simulink model "FullFMS_SIM_V0_1_7_R2026a"  (R2026a)
settings: Solver=FixedStepAuto  StopTime=inf  FixedStep=0.01  MaxStep=0.01  RelTol=1e-2
PreLoadFcn:
  | load("BUS_CONFIG_SIM.mat"); run("Param_SIM_V0_1_7.m")
libraries: opcualib x8
(part 1 of 2)
settings Model: SimulationMode=accelerator  PacingRate=0.100000  Creator=guilh  LastModifiedBy=gasie
settings SolverCC: ZeroCrossControl=DisableAll

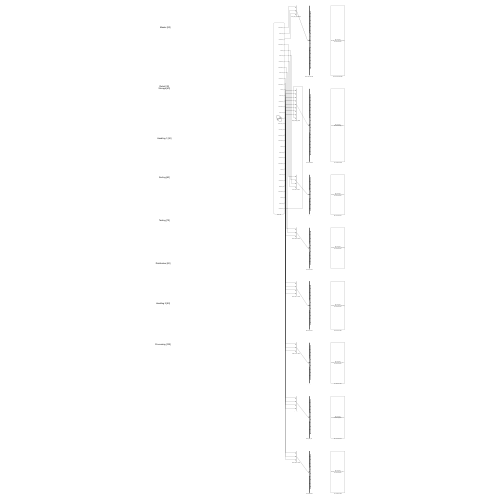
[thumbnail: Simulink's stored preview of the top-level diagram]
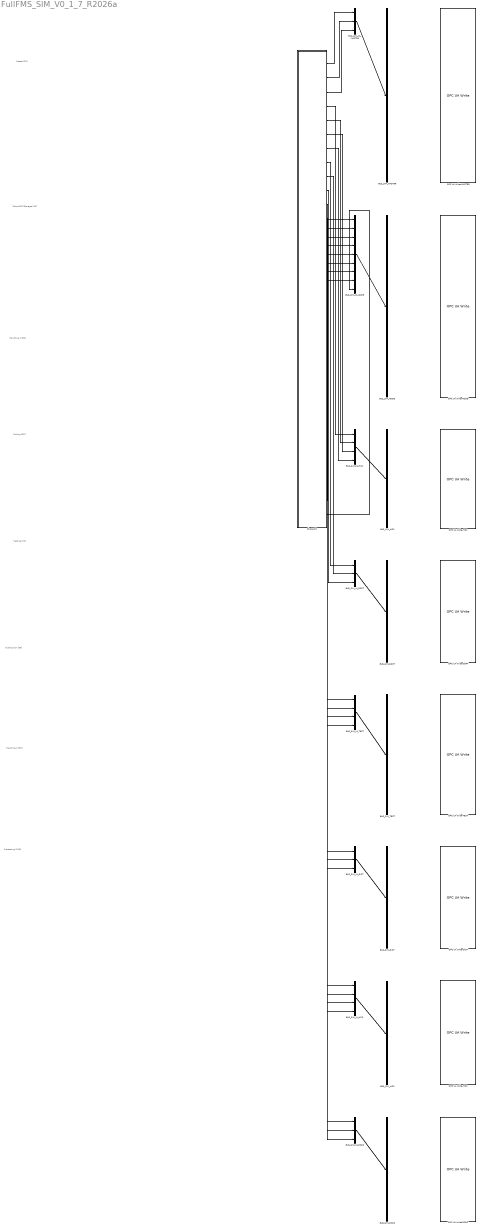
== system FullFMS_SIM_V0_1_7_R2026a ==
  note: Master [20]
  note: Robot [30]
      | Storage [40]
  note: Handling 1 [50]
  note: Sorting [60]
  note: Testing [70]
  note: Distribution [80]
  note: Handling 2 [90]
  note: Processing [100]
  BUS_SIM_DIST : BusSelector  OutputSignals=SimActuators_80.SA_80_Pist_Adv,SimActuators_80.SA_80_Suction_On,SimActuators_80.SA_80_Suction_Off,SimActuators_80.SA_80_Arm_2_Del,SimActuators_80.SA_80_Arm_2_Mag,SimActuators_80.SA_81_Led_Start,SimActuators_80.SA_81_Led_Reset,SimActuators_80.SA_81_Led_Extra1,SimActuators_80.SA_81_Led_Extra2,SimActuators_80.SA_81_Panel_O4,SimActuators_80.SA_81_Panel_O5,SimActuators_80.SA_81_Panel_O6,SimActuators_80.SA_81_Panel_O7,SimControl_80.SC_82_Profibus,SimControl_80.SC_83_RQ_Parts,SimControl_80.SC_85_Initialization,SimControl_80.SC_85_Start,SimControl_80.SC_85_Part_Del,SimControl_80.SC_85_Single,SimControl_80.SC_85_Part_Mag,SimControl_80.SC_85_Continuous,SimControl_80.SC_85_Counted,SimControl_80.SC_86_Mag_Parts,SimControl_80.SC_87_RQ_MParts,SimSensors_80.SS_80_Mag_Full,SimSensors_80.SS_80_Pist_Bck,SimSensors_80.SS_80_Pist_Fwd,SimSensors_80.SS_80_Part_Stuck,SimSensors_80.SS_80_Arm_Mag,SimSensors_80.SS_80_Arm_Del,SimSensors_80.SS_80_Mag_Empty,SimSensors_80.SS_81_Start,SimSensors_80.SS_81_Stop,SimSensors_80.SS_81_Key_Pos,SimSensors_80.SS_81_Reset,SimSensors_80.SS_81_Panel_I4,SimSensors_80.SS_81_Panel_I5,SimSensors_80.SS_81_Panel_I6,SimSensors_80.SS_81_Panel_I7
  BUS_SIM_HD1 : BusSelector  OutputSignals=SimActuators_50.SA_50_Claw_2_Del,SimActuators_50.SA_50_Claw_2_Cart,SimActuators_50.SA_50_Claw_Down,SimActuators_50.SA_50_Close_Claw,SimActuators_50.SA_51_Led_Start,SimActuators_50.SA_51_Led_Reset,SimActuators_50.SA_51_Led_Extra1,SimActuators_50.SA_51_Led_Extra2,SimActuators_50.SA_51_Panel_O4,SimActuators_50.SA_51_Panel_O5,SimActuators_50.SA_51_Panel_O6,SimActuators_50.SA_51_Panel_O7,SimASi_50.SR_53_SortCartID,SimASi_50.SR_54_Request,SimASi_50.SR_54_No_Cart,SimASi_50.SR_54_Cart_Full,SimASi_50.SR_54_CRoute_Out,SimASi_50.SR_54_CRoute_In,SimControl_50.SC_52_Profibus,SimControl_50.SC_55_Initialization,SimControl_50.SC_55_Start,SimControl_50.SC_55_PD_Sort,SimControl_50.SC_55_Cart2Del,SimSensors_50.SS_50_Part_Reserve,SimSensors_50.SS_50_Claw_Cart,SimSensors_50.SS_50_Claw_Del,SimSensors_50.SS_50_Claw_Reserve,SimSensors_50.SS_50_Claw_Low,SimSensors_50.SS_50_Claw_High,SimSensors_50.SS_50_Part_in_Claw,SimSensors_50.SS_51_Start,SimSensors_50.SS_51_Stop,SimSensors_50.SS_51_Key_Pos,SimSensors_50.SS_51_Reset,SimSensors_50.SS_51_Panel_I4,SimSensors_50.SS_51_Panel_I5,SimSensors_50.SS_51_Panel_I6,SimSensors_50.SS_51_Panel_I7
  BUS_SIM_HD2 : BusSelector  OutputSignals=SimActuators_90.SA_90_Claw_2_Cart,SimActuators_90.SA_90_Claw_2_Del,SimActuators_90.SA_90_Claw_Down,SimActuators_90.SA_90_Close_Claw,SimActuators_90.SA_91_Led_Start,SimActuators_90.SA_91_Led_Reset,SimActuators_90.SA_91_Led_Extra1,SimActuators_90.SA_91_Led_Extra2,SimActuators_90.SA_91_Panel_O4,SimActuators_90.SA_91_Panel_O5,SimActuators_90.SA_91_Panel_O6,SimActuators_90.SA_91_Panel_O7,SimASi_90.SR_93_ProcCartID,SimASi_90.SR_94_Request,SimASi_90.SR_94_No_Cart,SimASi_90.SR_94_Cart_Full,SimASi_90.SR_94_CRoute_Out,SimASi_90.SR_94_CRoute_In,SimControl_90.SC_92_Profibus,SimControl_90.SC_95_Initialization,SimControl_90.SC_95_Start,SimControl_90.SC_95_PD_Proc,SimControl_90.SC_95_Cart2Del,SimControl_90.SC_95_PD_Cart,SimControl_90.SC_95_Del2Cart,SimSensors_90.SS_90_Part_Reserve,SimSensors_90.SS_90_Claw_Del,SimSensors_90.SS_90_Claw_Cart,SimSensors_90.SS_90_Claw_Reserve,SimSensors_90.SS_90_Claw_Low,SimSensors_90.SS_90_Claw_High,SimSensors_90.SS_90_Part_in_Claw,SimSensors_90.SS_91_Start,SimSensors_90.SS_91_Stop,SimSensors_90.SS_91_Key_Pos,SimSensors_90.SS_91_Reset,SimSensors_90.SS_91_Panel_I4,SimSensors_90.SS_91_Panel_I5,SimSensors_90.SS_91_Panel_I6,SimSensors_90.SS_91_Panel_I7
  BUS_SIM_IN_DIST : BusCreator  Inputs=3  OutDataTypeStr=Bus: B_SIM_DIST  NonVirtualBus=on
  BUS_SIM_IN_HD1 : BusCreator  Inputs=4  OutDataTypeStr=Bus: B_SIM_HD1  NonVirtualBus=on
  BUS_SIM_IN_HD2 : BusCreator  Inputs=4  OutDataTypeStr=Bus: B_SIM_HD2  NonVirtualBus=on
  BUS_SIM_IN_MASTER : BusCreator  Inputs=3  OutDataTypeStr=Bus: B_SIM_MASTER  NonVirtualBus=on
  BUS_SIM_IN_NODE : BusCreator  Inputs=9  OutDataTypeStr=Bus: B_SIM_NODE  NonVirtualBus=on
  BUS_SIM_IN_PROC : BusCreator  Inputs=3  OutDataTypeStr=Bus: B_SIM_PROC  NonVirtualBus=on
  BUS_SIM_IN_SORT : BusCreator  Inputs=3  OutDataTypeStr=Bus: B_SIM_SORT  NonVirtualBus=on
  BUS_SIM_IN_TEST : BusCreator  Inputs=4  OutDataTypeStr=Bus: B_SIM_TEST  NonVirtualBus=on
  BUS_SIM_MASTER : BusSelector  OutputSignals=SimActuators_20.SA_20_Led_On,SimActuators_20.SA_20_Led_Off,SimActuators_20.SA_20_Conveyor,SimActuators_20.SA_24_Cart_Test,SimActuators_20.SA_25_Cart_Proc,SimActuators_20.SA_26_Cart_Visi,SimActuators_20.SA_27_Cart_Robo,SimActuators_20.SA_28_Cart_Stor,SimActuators_20.SA_29_Cart_Sort,SimControl_20.SC_21_MES_On,SimControl_20.SC_24_Request,SimControl_20.SC_24_CRoute_In,SimControl_20.SC_24_CartDel,SimControl_20.SC_24_CRoute_Out,SimControl_20.SC_25_Request,SimControl_20.SC_25_CRoute_In,SimControl_20.SC_25_CartDel,SimControl_20.SC_25_CRoute_Out,SimControl_20.SC_26_Request,SimControl_20.SC_26_CRoute_In,SimControl_20.SC_26_CartDel,SimControl_20.SC_26_CRoute_Out,SimControl_20.SC_27_Request,SimControl_20.SC_27_CRoute_In,SimControl_20.SC_27_CartDel,SimControl_20.SC_27_CRoute_Out,SimControl_20.SC_28_Request,SimControl_20.SC_28_CRoute_In,SimControl_20.SC_28_CartDel,SimControl_20.SC_28_CRoute_Out,SimControl_20.SC_29_Request,SimControl_20.SC_29_CRoute_In,SimControl_20.SC_29_CartDel,SimControl_20.SC_29_CRoute_Out,SimSensors_20.SS_20_On,SimSensors_20.SS_20_Off,SimSensors_20.SS_20_Controler_On,SimSensors_20.SS_24_Cart_Stat,SimSensors_20.SS_24_Cart_Next,SimSensors_20.SS_24_Optic,SimSensors_20.SS_24_Count,SimSensors_20.SS_24_Pist_Bck,SimSensors_20.SS_25_Cart_Stat,SimSensors_20.SS_25_Cart_Next,SimSensors_20.SS_25_Optic,SimSensors_20.SS_25_Count,SimSensors_20.SS_25_Pist_Bck,SimSensors_20.SS_26_Cart_Stat,SimSensors_20.SS_26_Cart_Next,SimSensors_20.SS_26_Optic,SimSensors_20.SS_26_Count,SimSensors_20.SS_26_Pist_Bck,SimSensors_20.SS_27_Cart_Stat,SimSensors_20.SS_27_Cart_Next,SimSensors_20.SS_27_Optic,SimSensors_20.SS_27_Count,SimSensors_20.SS_27_Pist_Bck,SimSensors_20.SS_28_Cart_Stat,SimSensors_20.SS_28_Cart_Next,SimSensors_20.SS_28_Optic,SimSensors_20.SS_28_Count,SimSensors_20.SS_28_Pist_Bck,SimSensors_20.SS_29_Cart_Stat,SimSensors_20.SS_29_Cart_Next,SimSensors_20.SS_29_Optic,SimSensors_20.SS_29_Count,SimSensors_20.SS_29_Pist_Bck
  BUS_SIM_NODE : BusSelector  OutputSignals=SimActuators_30.SA_30_Led_Start,SimActuators_30.SA_30_Led_Reset,SimActuators_30.SA_30_Led_Extra1,SimActuators_30.SA_30_Led_Extra2,SimActuators_30.SA_30_Spring_Cyl,SimActuators_30.SA_30_Cover_Cyl,SimASi_30.SR_32_RoboCartID,SimASi_30.SR_34_Request,SimASi_30.SR_34_No_Cart,SimASi_30.SR_34_Cart_Full,SimASi_30.SR_34_CRoute_Out,SimASi_30.SR_34_CRoute_In,SimControl_30.SC_30_Robot1,SimControl_30.SC_30_Robot2,SimControl_30.SC_35_Part_Del,SimSensors_30.SS_31_Start,SimSensors_30.SS_31_Stop,SimSensors_30.SS_31_Reset,SimSensors_30.SS_31_Part_in_Claw,SimSensors_30.SS_31_Orientation,SimSensors_30.SS_32_Sp_Cyl_Bck,SimSensors_30.SS_32_Sp_Cyl_Fwd,SimSensors_30.SS_32_Co_Cyl_Bck,SimSensors_30.SS_32_Co_Cyl_Fwd,SimSensors_30.SS_32_Sp_PickUp,SimSensors_30.SS_32_Co_PickUp,SimSensors_30.SS_32_CoMag_Empty,SimRFID_RFID.SID_Ant1_R_TagID,SimRFID_RFID.SID_Ant1_R_UserData,SimRFID_RFID.SID_Ant1_W_TagID,SimRFID_RFID.SID_Ant1_W_UserData,SimRFID_RFID.SID_Ant2_R_TagID,SimRFID_RFID.SID_Ant2_R_UserData,SimRFID_RFID.SID_Ant2_W_TagID,SimRFID_RFID.SID_Ant2_W_UserData,SimRFID_RFID.SID_Ant3_R_TagID,SimRFID_RFID.SID_Ant3_R_UserData,SimRFID_RFID.SID_Ant3_W_TagID,SimRFID_RFID.SID_Ant3_W_UserData,SimRFID_RFID.SID_Ant4_R_TagID,SimRFID_RFID.SID_Ant4_R_UserData,SimRFID_RFID.SID_Ant4_W_TagID,SimRFID_RFID.SID_Ant4_W_UserData,SimActuators_40.SA_41_Led_Start,SimActuators_40.SA_41_Led_Reset,SimActuators_40.SA_41_Led_Extra1,SimActuators_40.SA_41_Led_Extra2,SimActuators_40.SA_41_Panel_O4,SimActuators_40.SA_41_Panel_O5,SimActuators_40.SA_41_Panel_O6,SimActuators_40.SA_41_Panel_O7,SimASi_40.SR_43_StorCartID,SimASi_40.SR_44_Request,SimASi_40.SR_44_No_Cart,SimASi_40.SR_44_Cart_Full,SimASi_40.SR_44_CRoute_Out,SimASi_40.SR_44_CRoute_In,SimControl_40.SC_42_Profibus,SimControl_40.SC_45_Initialization,SimControl_40.SC_45_Start,SimControl_40.SC_45_StorePart,SimControl_40.SC_45_RetrievePart,SimSensors_40.SS_41_Start,SimSensors_40.SS_41_Stop,SimSensors_40.SS_41_Key_Pos,SimSensors_40.SS_41_Reset,SimSensors_40.SS_41_Panel_I4,SimSensors_40.SS_41_Panel_I5,SimSensors_40.SS_41_Panel_I6,SimSensors_40.SS_41_Panel_I7
  BUS_SIM_PROC : BusSelector  OutputSignals=SimActuators_100.SA_100_Drill_On,SimActuators_100.SA_100_RT_On,SimActuators_100.SA_100_Drill_Down,SimActuators_100.SA_100_Drill_Up,SimActuators_100.SA_100_Drill_Pin,SimActuators_100.SA_100_Test_Pin,SimActuators_100.SA_101_Led_Start,SimActuators_100.SA_101_Led_Reset,SimActuators_100.SA_101_Led_Extra1,SimActuators_100.SA_101_Led_Extra2,SimActuators_100.SA_101_Panel_O4,SimActuators_100.SA_101_Panel_O5,SimActuators_100.SA_101_Panel_O6,SimActuators_100.SA_101_Panel_O7,SimControl_100.SC_102_Profibus,SimControl_100.SC_103_RQ_Turns,SimControl_100.SC_105_Initialization,SimControl_100.SC_105_Start,SimControl_100.SC_105_Part_ready,SimControl_100.SC_105_Test,SimControl_100.SC_105_Test_Ok,SimControl_100.SC_105_TestDrill,SimControl_100.SC_105_Test_Fail,SimControl_100.SC_105_Rotation,SimControl_100.SC_106_RT_Counter,SimSensors_100.SS_100_PInit_Pos,SimSensors_100.SS_100_PDrill_Pos,SimSensors_100.SS_100_PTest_Pos,SimSensors_100.SS_100_SDrill_High,SimSensors_100.SS_100_SDrill_Low,SimSensors_100.SS_100_RT_Sensor,SimSensors_100.SS_100_PTest_Ok,SimSensors_100.SS_101_Start,SimSensors_100.SS_101_Stop,SimSensors_100.SS_101_Key_Pos,SimSensors_100.SS_101_Reset,SimSensors_100.SS_101_Panel_I4,SimSensors_100.SS_101_Panel_I5,SimSensors_100.SS_101_Panel_I6,SimSensors_100.SS_101_Panel_I7
  BUS_SIM_SORT : BusSelector  OutputSignals=SimActuators_60.SA_60_Conveyor,SimActuators_60.SA_60_P1,SimActuators_60.SA_60_P2,SimActuators_60.SA_60_Identify,SimActuators_60.SA_61_Led_Start,SimActuators_60.SA_61_Led_Reset,SimActuators_60.SA_61_Led_Extra1,SimActuators_60.SA_61_Led_Extra2,SimActuators_60.SA_61_Panel_O4,SimActuators_60.SA_61_Panel_O5,SimActuators_60.SA_61_Panel_O6,SimActuators_60.SA_61_Panel_O7,SimControl_60.SC_62_Profibus,SimControl_60.SC_65_Initialization,SimControl_60.SC_65_RBS_Output,SimControl_60.SC_65_ID_1,SimControl_60.SC_65_RSB_Output,SimControl_60.SC_65_ID_2,SimControl_60.SC_65_BRS_Output,SimControl_60.SC_65_Part_Sorted,SimControl_60.SC_65_BSR_Output,SimControl_60.SC_65_SRB_Output,SimControl_60.SC_65_SBR_Output,SimSensors_60.SS_60_SPart,SimSensors_60.SS_60_SInd,SimSensors_60.SS_60_SPhoto,SimSensors_60.SS_60_Part_Pass,SimSensors_60.SS_60_SL1_Bck,SimSensors_60.SS_60_SL1_Fwd,SimSensors_60.SS_60_SL2_Bck,SimSensors_60.SS_60_SL2_Fwd,SimSensors_60.SS_61_Start,SimSensors_60.SS_61_Stop,SimSensors_60.SS_61_Key_Pos,SimSensors_60.SS_61_Reset,SimSensors_60.SS_61_Panel_I4,SimSensors_60.SS_61_Panel_I5,SimSensors_60.SS_61_Panel_I6,SimSensors_60.SS_61_Panel_I7
  BUS_SIM_TEST : BusSelector  OutputSignals=SimActuators_70.SA_70_Elev_Down,SimActuators_70.SA_70_Elev_Up,SimActuators_70.SA_70_Eject_Part,SimActuators_70.SA_70_Air_On,SimActuators_70.SA_71_Led_Start,SimActuators_70.SA_71_Led_Reset,SimActuators_70.SA_71_Led_Extra1,SimActuators_70.SA_71_Led_Extra2,SimActuators_70.SA_71_Panel_O4,SimActuators_70.SA_71_Panel_O5,SimActuators_70.SA_71_Panel_O6,SimActuators_70.SA_71_Panel_O7,SimASi_70.SR_73_TestCartID,SimASi_70.SR_74_Request,SimASi_70.SR_74_No_Cart,SimASi_70.SR_74_Cart_Full,SimASi_70.SR_74_CRoute_Out,SimASi_70.SR_74_CRoute_In,SimControl_70.SC_72_Profibus,SimControl_70.SC_75_Initialization,SimControl_70.SC_75_RQ_Delivery1,SimControl_70.SC_75_ID_Delivery1,SimControl_70.SC_75_RQ_Delivery2,SimControl_70.SC_75_ID_Delivery2,SimControl_70.SC_75_Identified,SimControl_70.SC_75_Part_Del,SimControl_70.SC_75_Requested,SimControl_70.SC_75_RQ_Part_Del,SimControl_70.SC_75_RQ_Wrong,SimControl_70.SC_75_Identified80,SimControl_70.SC_75_Requested80,SimSensors_70.SS_70_SInductive,SimSensors_70.SS_70_SPart,SimSensors_70.SS_70_SStation,SimSensors_70.SS_70_SPart_Height,SimSensors_70.SS_70_Elev_High,SimSensors_70.SS_70_Elev_Low,SimSensors_70.SS_70_Pist_Bck,SimSensors_70.SS_71_Start,SimSensors_70.SS_71_Stop,SimSensors_70.SS_71_Key_Pos,SimSensors_70.SS_71_Reset,SimSensors_70.SS_71_Panel_I4,SimSensors_70.SS_71_Panel_I5,SimSensors_70.SS_71_Panel_I6,SimSensors_70.SS_71_Panel_I7
  Chart_SIM : Stateflow chart  TreatAsAtomicUnit=on
  OPC UA Write-DIST : opcualib/OPC UA Write  SelectedServer=AAS OPC Distribution (200.145.26.206)  ServerList=AAS OPC Distribution (200.145.26.206)  NodeList={}  OnWriteFailure=Error and stop  SampleTime=-1
  OPC UA Write-HD1 : opcualib/OPC UA Write  SelectedServer=AAS OPC Handling1 (200.145.26.203)  ServerList=AAS OPC Handling1 (200.145.26.203)  NodeList={}  OnWriteFailure=Error and stop  SampleTime=-1
  OPC UA Write-HD2 : opcualib/OPC UA Write  SelectedServer=AAS OPC Handling2 (200.145.26.207)  ServerList=AAS OPC Handling2 (200.145.26.207)  NodeList={}  OnWriteFailure=Error and stop  SampleTime=-1
  OPC UA Write-MASTER : opcualib/OPC UA Write  SelectedServer=AAS OPC Master (200.145.26.202)  ServerList=AAS OPC Master (200.145.26.202)  NodeList={}  OnWriteFailure=Error and stop  SampleTime=-1
  OPC UA Write-NODE : opcualib/OPC UA Write  SelectedServer=AAS Server Robot+Storage (200.145.26.213)  ServerList=AAS Server Robot+Storage (200.145.26.213)  NodeList={}  OnWriteFailure=Error and stop  SampleTime=-1
  OPC UA Write-PROC : opcualib/OPC UA Write  SelectedServer=AAS OPC Processing (200.145.26.208)  ServerList=AAS OPC Processing (200.145.26.208)  NodeList={}  OnWriteFailure=Error and stop  SampleTime=-1
  OPC UA Write-SORT : opcualib/OPC UA Write  SelectedServer=AAS OPC Sorting (200.145.26.204)  ServerList=AAS OPC Sorting (200.145.26.204)  NodeList={}  OnWriteFailure=Error and stop  SampleTime=-1
  OPC UA Write-TEST : opcualib/OPC UA Write  SelectedServer=AAS OPC Testing (200.145.26.205)  ServerList=AAS OPC Testing (200.145.26.205)  NodeList={}  OnWriteFailure=Error and stop  SampleTime=-1
  wires:
  BUS_SIM_IN_MASTER/1 -> BUS_SIM_MASTER/1
  BUS_SIM_IN_NODE/1 -> BUS_SIM_NODE/1
  BUS_SIM_IN_HD1/1 -> BUS_SIM_HD1/1
  BUS_SIM_IN_SORT/1 -> BUS_SIM_SORT/1
  BUS_SIM_IN_TEST/1 -> BUS_SIM_TEST/1
  BUS_SIM_IN_DIST/1 -> BUS_SIM_DIST/1
  BUS_SIM_IN_HD2/1 -> BUS_SIM_HD2/1
  BUS_SIM_IN_PROC/1 -> BUS_SIM_PROC/1
  Chart_SIM/1(SimActuators_20) -> BUS_SIM_IN_MASTER/1
  Chart_SIM/2(SimControl_20) -> BUS_SIM_IN_MASTER/2
  Chart_SIM/3(SimSensors_20) -> BUS_SIM_IN_MASTER/3
  Chart_SIM/4(SimActuators_50) -> BUS_SIM_IN_HD1/1
  Chart_SIM/5(SimASi_50) -> BUS_SIM_IN_HD1/2
  Chart_SIM/6(SimControl_50) -> BUS_SIM_IN_HD1/3
  Chart_SIM/7(SimSensors_50) -> BUS_SIM_IN_HD1/4
  Chart_SIM/8(SimActuators_60) -> BUS_SIM_IN_SORT/1
  Chart_SIM/9(SimControl_60) -> BUS_SIM_IN_SORT/2
  Chart_SIM/10(SimSensors_60) -> BUS_SIM_IN_SORT/3
  Chart_SIM/11(SimActuators_70) -> BUS_SIM_IN_TEST/1
  Chart_SIM/12(SimASi_70) -> BUS_SIM_IN_TEST/2
  Chart_SIM/13(SimControl_70) -> BUS_SIM_IN_TEST/3
  Chart_SIM/14(SimSensors_70) -> BUS_SIM_IN_TEST/4
  Chart_SIM/15(SimActuators_80) -> BUS_SIM_IN_DIST/1
  Chart_SIM/16(SimControl_80) -> BUS_SIM_IN_DIST/2
  Chart_SIM/17(SimSensors_80) -> BUS_SIM_IN_DIST/3
  Chart_SIM/18(SimActuators_100) -> BUS_SIM_IN_PROC/1
  Chart_SIM/19(SimControl_100) -> BUS_SIM_IN_PROC/2
  Chart_SIM/20(SimSensors_100) -> BUS_SIM_IN_PROC/3
  Chart_SIM/21(SimActuators_90) -> BUS_SIM_IN_HD2/1
  Chart_SIM/22(SimASi_90) -> BUS_SIM_IN_HD2/2
  Chart_SIM/23(SimControl_90) -> BUS_SIM_IN_HD2/3
  Chart_SIM/24(SimSensors_90) -> BUS_SIM_IN_HD2/4
  Chart_SIM/25(SimActuators_30) -> BUS_SIM_IN_NODE/1
  Chart_SIM/26(SimASi_30) -> BUS_SIM_IN_NODE/2
  Chart_SIM/27(SimControl_30) -> BUS_SIM_IN_NODE/3
  Chart_SIM/28(SimSensors_30) -> BUS_SIM_IN_NODE/4
  Chart_SIM/29(SimRFID_RFID) -> BUS_SIM_IN_NODE/5
  Chart_SIM/30(SimActuators_40) -> BUS_SIM_IN_NODE/6
  Chart_SIM/31(SimASi_40) -> BUS_SIM_IN_NODE/7
  Chart_SIM/32(SimControl_40) -> BUS_SIM_IN_NODE/8
  Chart_SIM/33(SimSensors_40) -> BUS_SIM_IN_NODE/9
